simulink library "tandem_tiltwing_lib"  (R2018b)
settings: Solver=VariableStepAuto  StartTime=0.0  StopTime=10.0  RelTol=1e-3
undefined symbols (not defined in the file or in its folder): envir, euler2Quat, tiltwing
libraries: propulsion_lib x4, actuators_lib x3, simple_wing_lib x2, simpleFuselage_lib x1, ground_lib x1, rigidBody_lib x1
settings Model: Creator=Ybeyer  LastModifiedBy=yannic
settings SFSimCC: SimUseLocalCustomCode=off
settings RTWCC: RTWUseLocalCustomCode=off
settings CodeAppCC: StateflowObjectComments=on

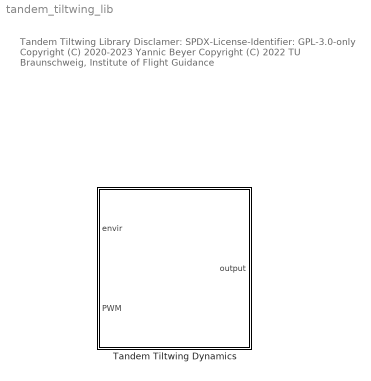
== system tandem_tiltwing_lib ==
  note: Tandem Tiltwing Library
      |
      | Disclamer:
      | SPDX-License-Identifier: GPL-3.0-only
      |
      | Copyright (C) 2020-2023 Yannic Beyer
      | Copyright (C) 2022 TU Braunschweig, Institute of Flight Guidance
  Tandem Tiltwing Dynamics : Subsystem  mask{tiltwing=tiltwing}
      mask prompts: tiltwing "tiltwing struct"
      mask DialogControl DescGroupVar Prompt: Tandem Tiltwing Dynamics
      mask DialogControl DescTextVar Prompt: For initializing the tiltwing struct see tandemTiltwingLoadParams.m

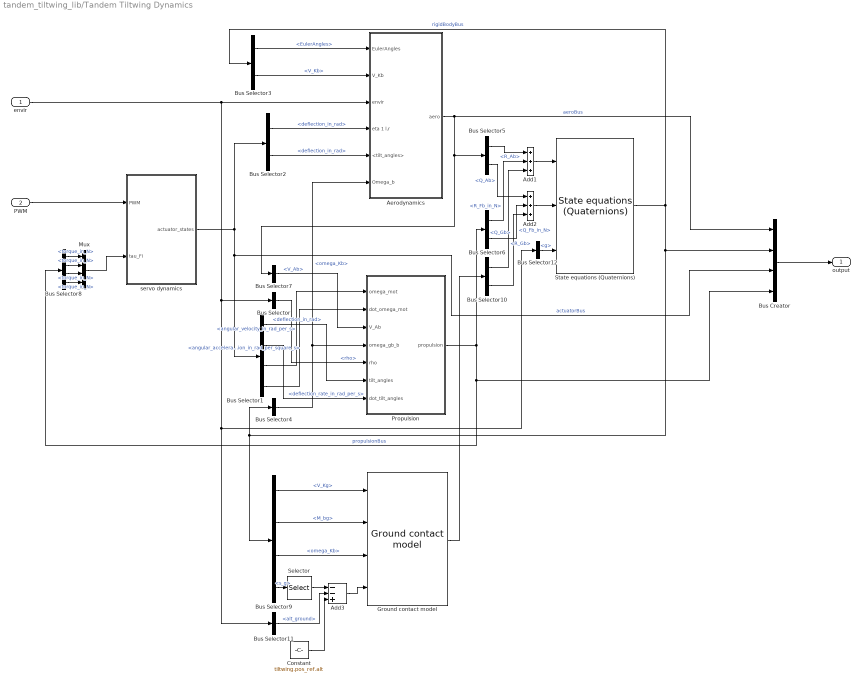
== system tandem_tiltwing_lib/Tandem Tiltwing Dynamics ==
  envir : Inport
  PWM : Inport  Port=2
  Add1 : Sum  Inputs=3
  Add2 : Sum  Inputs=3
  Add3 : Sum  Inputs=--+
  Aerodynamics : Subsystem
  Bus Creator : BusCreator  Inputs=4
  Bus Selector : BusSelector  OutputSignals=atmosphereBus.rho
  Bus Selector1 : BusSelector  OutputSignals=tilt_servos.deflection_in_rad,elevons.deflection_rate_in_rad_per_s,motors.angular_velocity_in_rad_per_s,motors.angular_acceleration_in_rad_per_square_s
  Bus Selector10 : BusSelector  OutputSignals=forces_and_moments.R_Gb,forces_and_moments.Q_Gb
  Bus Selector11 : BusSelector  OutputSignals=alt_ground
  Bus Selector12 : BusSelector  OutputSignals=g
  Bus Selector2 : BusSelector  OutputSignals=elevons.deflection_in_rad,tilt_servos.deflection_in_rad
  Bus Selector3 : BusSelector  OutputSignals=EulerAngles,V_Kb
  Bus Selector4 : BusSelector  OutputSignals=omega_Kb
  Bus Selector5 : BusSelector  OutputSignals=cg aerodynamics.R_Ab,cg aerodynamics.Q_Ab
  Bus Selector6 : BusSelector  OutputSignals=R_Fb_in_N,Q_Fb_in_N
  Bus Selector7 : BusSelector  OutputSignals=cg aerodynamics.aeroAxes.V_Ab
  Bus Selector8 : BusSelector  OutputSignals=propeller_1.torque_in_N,propeller_2.torque_in_N,propeller_3.torque_in_N,propeller_4.torque_in_N
  Bus Selector9 : BusSelector  OutputSignals=V_Kg,M_bg,omega_Kb,s_g
  Constant : Constant  Value=tiltwing.pos_ref.alt  VectorParams1D=off
  Ground contact model : ground_lib/Ground contact model  m=tiltwing.body.m  a_max=30  xyz_c_hit=tiltwing.config.collision_points_c  xyz_c_cg=tiltwing.config.xyz_c_cg  ground_softness_param=1e-5  k_h=1000  k_dot_h=100  mu=1  k_V=10
      settings: SourceProductName=LADAC
  Mux : Mux
  Propulsion : Subsystem
  Selector : Selector  InputPortWidth=3  IndexOptions=Index vector (dialog)  Indices=3  OutputSizes=1
  State equations (Quaternions) : rigidBody_lib/State equations (Quaternions)  m=tiltwing.body.m  I=tiltwing.body.I  is_g_checked=on  g=envir.g  omega_Kb_0=[ tiltwing.ic.p; tiltwing.ic.q; tiltwing.ic.r ]  q_bg_0=euler2Quat( [ tiltwing.ic.Phi; tiltwing.ic.Theta; tiltwing.ic.Psi ] )  V_Kb_0=[ tiltwing.ic.u; tiltwing.ic.v ; tiltwing.ic.w ]  s_g_0=[ tiltwing.ic.x; tiltwing.ic.y; tiltwing.ic.z ]
      settings: SourceProductName=LADAC
  servo dynamics : Subsystem
  output : Outport
  wires:
  PWM/1 -> servo dynamics/1(PWM)
  Bus Selector/1 -> Propulsion/5(rho)  "<rho>"
  servo dynamics/1(actuator_states) -> Bus Creator/3, Bus Selector1/1, Bus Selector2/1  "actuatorBus"
  Bus Selector1/1 -> Propulsion/6(tilt_angles)  "<deflection_in_rad>"
  Bus Selector1/3 -> Propulsion/1(omega_mot)  "<angular_velocity_in_rad_per_s>"
  Bus Selector1/4 -> Propulsion/2(dot_omega_mot)  "<angular_acceleration_in_rad_per_square_s>"
  Bus Selector2/1 -> Aerodynamics/4(eta 1 l,r)  "<deflection_in_rad>"
  Bus Selector2/2 -> Aerodynamics/5(<tilt_angles>)  "<deflection_in_rad>"
  State equations (Quaternions)/1 -> Bus Selector3/1, Bus Selector9/1, Bus Selector4/1, Bus Creator/2  "rigidBodyBus"
  Bus Selector3/2 -> Aerodynamics/2(V_Kb)  "<V_Kb>"
  Bus Selector3/1 -> Aerodynamics/1("EulerAngles ")  "<EulerAngles>"
  Bus Selector4/1 -> Propulsion/4("omega_gb_b "), Aerodynamics/6(Omega_b)  "<omega_Kb>"
  Bus Selector5/1 -> Add1/1  "<R_Ab>"
  Bus Selector5/2 -> Add2/1  "<Q_Ab>"
  Aerodynamics/1(aero) -> Bus Creator/1, Bus Selector5/1, Bus Selector7/1  "aeroBus"
  Bus Selector6/2 -> Add2/2  "<Q_Fb_in_N>"
  Bus Selector6/1 -> Add1/2  "<R_Fb_in_N>"
  Propulsion/1(propulsion) -> Bus Creator/4, Bus Selector8/1, Bus Selector6/1  "propulsionBus"
  Bus Selector7/1 -> Propulsion/3(V_Ab)  "<V_Ab>"
  Bus Selector9/1 -> Ground contact model/1  "<V_Kg>"
  Add1/1 -> State equations (Quaternions)/1
  Add2/1 -> State equations (Quaternions)/2
  Bus Selector9/3 -> Ground contact model/3  "<omega_Kb>"
  Bus Selector9/2 -> Ground contact model/2  "<M_bg>"
  Ground contact model/1 -> Bus Selector10/1
  Bus Selector10/1 -> Add1/3  "<R_Gb>"
  Bus Selector9/4 -> Selector/1  "<s_g>"
  Add3/1 -> Ground contact model/4
  Bus Selector11/1 -> Add3/2  "<alt_ground>"
  Selector/1 -> Add3/1
  Bus Selector10/2 -> Add2/3  "<Q_Gb>"
  Bus Selector1/2 -> Propulsion/7(dot_tilt_angles)  "<deflection_rate_in_rad_per_s>"
  Bus Selector8/4 -> Mux/4  "<torque_in_N>"
  Bus Selector8/3 -> Mux/3  "<torque_in_N>"
  Bus Selector8/2 -> Mux/2  "<torque_in_N>"
  Bus Selector8/1 -> Mux/1  "<torque_in_N>"
  Mux/1 -> servo dynamics/2(tau_Fi)
  Bus Creator/1 -> output/1
  envir/1 -> Aerodynamics/3(envir), Bus Selector/1, Bus Selector11/1, Bus Selector12/1
  Constant/1 -> Add3/3
  Bus Selector12/1 -> State equations (Quaternions)/3  "<g>"

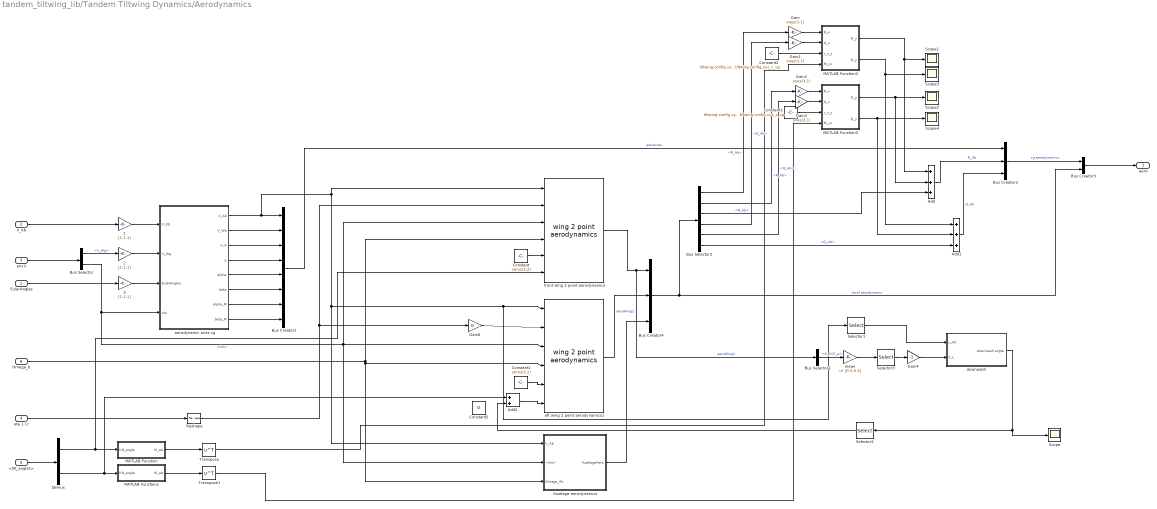
== system tandem_tiltwing_lib/Tandem Tiltwing Dynamics/Aerodynamics ==
  "EulerAngles " : Inport
  V_Kb : Inport  Port=2
  envir : Inport  Port=3
  eta 1 l,r : Inport  Port=4
  <tilt_angles> : Inport  Port=5
  Omega_b : Inport  Port=6
  1 : Gain  Gain=[1;1;1]
  2 : Gain  Gain=[1;1;1]  OutDataTypeStr=double
  3 : Gain  Gain=[1;1;1]
  Add : Sum  Inputs=+++
  Add1 : Sum  Inputs=+++
  Add2 : Sum
  Bus Creator1 : BusCreator  Inputs=8
  Bus Creator2 : BusCreator  Inputs=3
  Bus Creator3 : BusCreator  Inputs=2
  Bus Creator4 : BusCreator  Inputs=3
  Bus Selector : BusSelector  OutputSignals=windBus.V_Wg,atmosphereBus.rho
  Bus Selector1 : BusSelector  OutputSignals=dynamics.C_XYZ_a
  Bus Selector2 : BusSelector  OutputSignals=aeroWing1.dynamics.R_Ab,aeroWing2.dynamics.R_Ab,aeroFuselage.dynamics.R_Ab,aeroWing1.dynamics.Q_Ab,aeroWing2.dynamics.Q_Ab,aeroFuselage.dynamics.Q_Ab
  Constant : Constant  Value=zeros(3,2)
  Constant1 : Constant  Value=zeros(3,2)
  Constant2 : Constant  Value=tiltwing.config.xyz_c_tp1-tiltwing.config.xyz_c_cg
  Constant3 : Constant  Value=tiltwing.config.xyz_c_tp2-tiltwing.config.xyz_c_cg
  Constant5 : Constant  Value=0
  Demux : Demux  Outputs=2
  Gain{,1..3} (4 alike) : Gain  Gain=ones(3,1)
  Gain4 : Gain  Gain=-1
  Gain6 : Gain  Gain=0
  MATLAB Function : MATLAB Function  TreatAsAtomicUnit=on
  MATLAB Function1 : MATLAB Function  TreatAsAtomicUnit=on
  MATLAB Function2 : MATLAB Function  TreatAsAtomicUnit=on
  MATLAB Function3 : MATLAB Function  TreatAsAtomicUnit=on
  Reshape : Reshape  OutputDimensionality=Row vector (2-D)
  Scope{,1..4} (5 alike) : Scope
  Selector1 : Selector  InputPortWidth=3  IndexOptions=Index vector (dialog)  Indices=1  OutputSizes=1
  Selector2 : Selector  InputPortWidth=1  IndexOptions=Index vector (dialog)  Indices=1  OutputSizes=1
  Selector3 : Selector  InputPortWidth=3  IndexOptions=Index vector (dialog)  Indices=3  OutputSizes=1
  Transpose : Math  Operator=transpose  SaturateOnIntegerOverflow=on
  Transpose1 : Math  Operator=transpose  SaturateOnIntegerOverflow=on
  aerodynamic axes cg : MATLAB Function  TreatAsAtomicUnit=on
  aft wing 2 point aerodynamics1 : simple_wing_lib/wing 2 point aerodynamics  wingStruct=tiltwing.aero.wing_2  xyz_wing_c=tiltwing.config.xyz_c_tp2  xyz_cg_c=tiltwing.config.xyz_c_cg
      settings: SourceProductName=LADAC
  downwash : Subsystem
  front wing 2 point aerodynamics : simple_wing_lib/wing 2 point aerodynamics  wingStruct=tiltwing.aero.wing_1  xyz_wing_c=tiltwing.config.xyz_c_tp1  xyz_cg_c=tiltwing.config.xyz_c_cg
      settings: SourceProductName=LADAC
  fuselage aerodynamics : Subsystem
  mean : Gain  Gain=[0.5;0.5]  Multiplication=Matrix(u*K)
  aero : Outport
  wires:
  envir/1 -> Bus Selector/1
  Bus Selector/1 -> 2/1  "<V_Wg>"
  2/1 -> aerodynamic axes cg/2(V_Wg)
  "EulerAngles "/1 -> 3/1
  1/1 -> aerodynamic axes cg/1(V_Kb)
  V_Kb/1 -> 1/1
  3/1 -> aerodynamic axes cg/3(EulerAngles)
  Bus Selector/2 -> aft wing 2 point aerodynamics1/3, fuselage aerodynamics/2(<rho>), front wing 2 point aerodynamics/3, aerodynamic axes cg/4(rho)  "<rho>"
  eta 1 l,r/1 -> Reshape/1
  aerodynamic axes cg/2(V_Wb) -> Bus Creator1/2
  aerodynamic axes cg/3(V_A) -> Bus Creator1/3
  aerodynamic axes cg/4(q) -> Bus Creator1/4
  aerodynamic axes cg/5(alpha) -> Bus Creator1/5
  aerodynamic axes cg/6(beta) -> Bus Creator1/6
  aerodynamic axes cg/7(alpha_M) -> Bus Creator1/7
  aerodynamic axes cg/8(beta_M) -> Bus Creator1/8
  Bus Creator1/1 -> Bus Creator2/1  "aeroAxes"
  Bus Creator2/1 -> Bus Creator3/1  "cg aerodynamics"
  Bus Creator4/1 -> Bus Creator3/2, Bus Selector2/1  "local aerodynamic"
  Bus Creator3/1 -> aero/1
  front wing 2 point aerodynamics/1 -> Bus Selector1/1, Bus Creator4/1  "aeroWing1"
  aft wing 2 point aerodynamics1/1 -> Bus Creator4/2  "aeroWing2"
  fuselage aerodynamics/1(fuselageAero) -> Bus Creator4/3
  Bus Selector2/3 -> Add/3  "<R_Ab>"
  Bus Selector2/2 -> Gain2/1  "<R_Ab>"
  Bus Selector2/1 -> Gain/1  "<R_Ab>"
  Bus Selector2/6 -> Add1/3  "<Q_Ab>"
  Bus Selector2/5 -> Gain3/1  "<Q_Ab>"
  Bus Selector2/4 -> Gain1/1  "<Q_Ab>"
  Add/1 -> Bus Creator2/2  "R_Ab"
  Add1/1 -> Bus Creator2/3  "Q_Ab"
  Constant/1 -> front wing 2 point aerodynamics/5
  Constant1/1 -> aft wing 2 point aerodynamics1/5
  <tilt_angles>/1 -> Demux/1
  Demux/1 -> MATLAB Function/1(tilt_angle), front wing 2 point aerodynamics/6
  Demux/2 -> MATLAB Function1/1(tilt_angle), Add2/1
  aerodynamic axes cg/1(V_Ab) -> Bus Creator1/1, front wing 2 point aerodynamics/1, fuselage aerodynamics/1(V_Ab), Selector1/1, aft wing 2 point aerodynamics1/1
  MATLAB Function1/1(M_wb) -> Transpose1/1
  MATLAB Function/1(M_wb) -> Transpose/1
  Omega_b/1 -> front wing 2 point aerodynamics/4, fuselage aerodynamics/3(Omega_Ab), aft wing 2 point aerodynamics1/4
  Constant2/1 -> MATLAB Function2/3(r_x_y)
  Constant3/1 -> MATLAB Function3/3(r_x_y)
  MATLAB Function2/1(R_y) -> Scope1/1, Add/1
  MATLAB Function3/1(R_y) -> Scope2/1, Add/2
  MATLAB Function2/2(Q_y) -> Scope3/1, Add1/1
  MATLAB Function3/2(Q_y) -> Add1/2, Scope4/1
  Gain/1 -> MATLAB Function2/1(R_x)
  Gain1/1 -> MATLAB Function2/2(Q_x)
  Gain2/1 -> MATLAB Function3/1(R_x)
  Gain3/1 -> MATLAB Function3/2(Q_x)
  Transpose/1 -> MATLAB Function2/4(M_yx)
  Transpose1/1 -> MATLAB Function3/4(M_yx)
  Add2/1 -> aft wing 2 point aerodynamics1/6
  downwash/1(downwash angle) -> Selector2/1, Scope/1
  Gain4/1 -> downwash/2(C_L)
  Selector1/1 -> downwash/1(u_Ab)
  Bus Selector1/1 -> mean/1  "<C_XYZ_a>"
  Selector2/1 -> Add2/2
  Selector3/1 -> Gain4/1
  mean/1 -> Selector3/1
  Reshape/1 -> Gain6/1, front wing 2 point aerodynamics/2
  Gain6/1 -> aft wing 2 point aerodynamics1/2

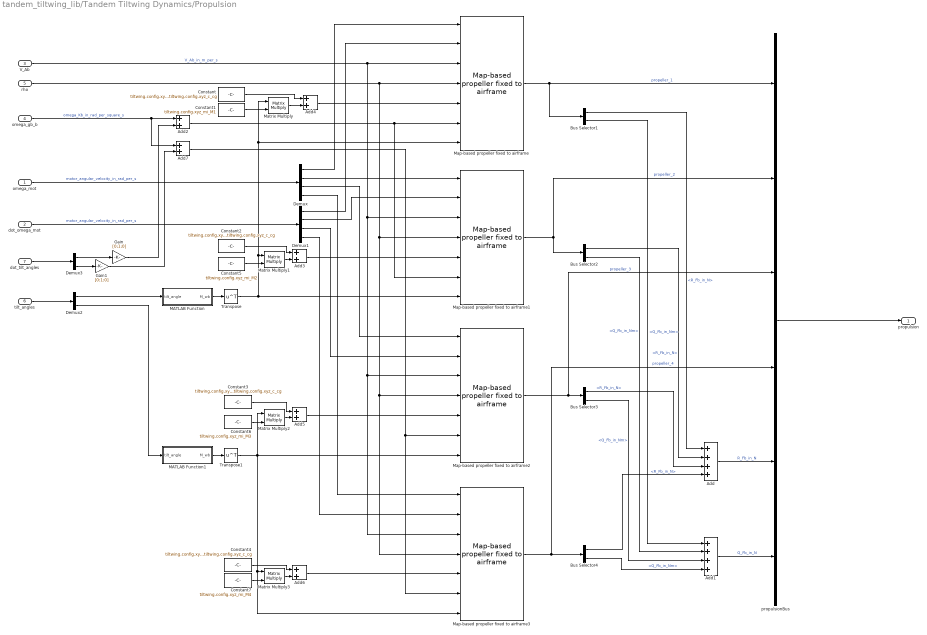
== system tandem_tiltwing_lib/Tandem Tiltwing Dynamics/Propulsion ==
  omega_mot : Inport  OutDataTypeStr=double  PortDimensions=4  SampleTime=0
  dot_omega_mot : Inport  Port=2  OutDataTypeStr=double  PortDimensions=4  SampleTime=0
  V_Ab : Inport  Port=3  OutDataTypeStr=double  PortDimensions=3  SampleTime=0
  "omega_gb_b " : Inport  Port=4  OutDataTypeStr=double  PortDimensions=3  SampleTime=0
  rho : Inport  Port=5  OutDataTypeStr=double  PortDimensions=1
  tilt_angles : Inport  Port=6
  dot_tilt_angles : Inport  Port=7
  Add : Sum  Inputs=4
  Add1 : Sum  Inputs=4
  Add{2..7} (6 alike) : Sum
  Bus Selector{1..4} (4 alike) : BusSelector  OutputSignals=R_Fb_in_N,Q_Fb_in_Nm
  Constant : Constant  Value=tiltwing.config.xyz_c_tp1-tiltwing.config.xyz_c_cg
  Constant1 : Constant  Value=tiltwing.config.xyz_mi_M1
  Constant2 : Constant  Value=tiltwing.config.xyz_c_tp1-tiltwing.config.xyz_c_cg
  Constant3 : Constant  Value=tiltwing.config.xyz_c_tp2-tiltwing.config.xyz_c_cg
  Constant4 : Constant  Value=tiltwing.config.xyz_c_tp2-tiltwing.config.xyz_c_cg
  Constant5 : Constant  Value=tiltwing.config.xyz_mi_M2
  Constant6 : Constant  Value=tiltwing.config.xyz_mi_M3
  Constant7 : Constant  Value=tiltwing.config.xyz_mi_M4
  Demux : Demux
  Demux1 : Demux
  Demux2 : Demux  Outputs=2
  Demux3 : Demux  Outputs=2
  Gain : Gain  Gain=[0;1;0]
  Gain1 : Gain  Gain=[0;1;0]
  MATLAB Function : MATLAB Function  TreatAsAtomicUnit=on
  MATLAB Function1 : MATLAB Function  TreatAsAtomicUnit=on
  Map-based propeller fixed to airframe : propulsion_lib/Map-based propeller fixed to airframe  prop_map_fit=prop.map_fit  I_prop=tiltwing.prop.I  rotation_orientation=tiltwing.config.propDir(1)
      settings: SourceProductName=LADAC
  Map-based propeller fixed to airframe1 : propulsion_lib/Map-based propeller fixed to airframe  prop_map_fit=prop.map_fit  I_prop=tiltwing.prop.I  rotation_orientation=tiltwing.config.propDir(2)
      settings: SourceProductName=LADAC
  Map-based propeller fixed to airframe2 : propulsion_lib/Map-based propeller fixed to airframe  prop_map_fit=prop.map_fit  I_prop=tiltwing.prop.I  rotation_orientation=tiltwing.config.propDir(3)
      settings: SourceProductName=LADAC
  Map-based propeller fixed to airframe3 : propulsion_lib/Map-based propeller fixed to airframe  prop_map_fit=prop.map_fit  I_prop=tiltwing.prop.I  rotation_orientation=tiltwing.config.propDir(4)
      settings: SourceProductName=LADAC
  Matrix Multiply{,1..3} (4 alike) : Product  Multiplication=Matrix(*)
  Transpose : Math  Operator=transpose  SaturateOnIntegerOverflow=on
  Transpose1 : Math  Operator=transpose  SaturateOnIntegerOverflow=on
  propulsionBus : BusCreator  Inputs=6
  propulsion : Outport  SampleTime=0
  wires:
  Demux1/1 -> Map-based propeller fixed to airframe/2
  V_Ab/1 -> Map-based propeller fixed to airframe3/3, Map-based propeller fixed to airframe2/3, Map-based propeller fixed to airframe1/3, Map-based propeller fixed to airframe/3  "V_Ab_in_m_per_s"
  Bus Selector1/1 -> Add/1  "<R_Fb_in_N>"
  Add4/1 -> Map-based propeller fixed to airframe/5
  Bus Selector2/1 -> Add/2  "<R_Fb_in_N>"
  Bus Selector1/2 -> Add1/1  "<Q_Fb_in_Nm>"
  Demux1/3 -> Map-based propeller fixed to airframe2/2
  Demux1/4 -> Map-based propeller fixed to airframe3/2
  Bus Selector4/1 -> Add/4  "<R_Fb_in_N>"
  Bus Selector3/2 -> Add1/3  "<Q_Fb_in_Nm>"
  Demux1/2 -> Map-based propeller fixed to airframe1/2
  Demux/1 -> Map-based propeller fixed to airframe/1
  Add3/1 -> Map-based propeller fixed to airframe1/5
  Map-based propeller fixed to airframe3/1 -> Bus Selector4/1, propulsionBus/4  "propeller_4"
  propulsionBus/1 -> propulsion/1
  Bus Selector4/2 -> Add1/4  "<Q_Fb_in_Nm>"
  Demux/2 -> Map-based propeller fixed to airframe1/1
  Map-based propeller fixed to airframe1/1 -> Bus Selector2/1, propulsionBus/2  "propeller_2"
  Bus Selector3/1 -> Add/3  "<R_Fb_in_N>"
  Transpose1/1 -> Map-based propeller fixed to airframe2/7, Matrix Multiply3/1, Map-based propeller fixed to airframe3/7, Matrix Multiply2/1
  Add/1 -> propulsionBus/5  "R_Fb_in_N"
  Add2/1 -> Map-based propeller fixed to airframe1/6, Map-based propeller fixed to airframe/6
  Add5/1 -> Map-based propeller fixed to airframe2/5
  rho/1 -> Map-based propeller fixed to airframe3/4, Map-based propeller fixed to airframe2/4, Map-based propeller fixed to airframe1/4, Map-based propeller fixed to airframe/4
  Map-based propeller fixed to airframe2/1 -> propulsionBus/3, Bus Selector3/1  "propeller_3"
  Demux/3 -> Map-based propeller fixed to airframe2/1
  Transpose/1 -> Matrix Multiply1/1, Matrix Multiply/1, Map-based propeller fixed to airframe/7, Map-based propeller fixed to airframe1/7
  Bus Selector2/2 -> Add1/2  "<Q_Fb_in_Nm>"
  Map-based propeller fixed to airframe/1 -> propulsionBus/1, Bus Selector1/1  "propeller_1"
  Add1/1 -> propulsionBus/6  "Q_Fb_in_N"
  Add6/1 -> Map-based propeller fixed to airframe3/5
  Demux/4 -> Map-based propeller fixed to airframe3/1
  omega_mot/1 -> Demux/1  "motor_angular_velocity_in_rad_per_s"
  dot_omega_mot/1 -> Demux1/1  "motor_angular_velocity_in_rad_per_s"
  MATLAB Function/1(M_wb) -> Transpose/1
  tilt_angles/1 -> Demux2/1
  Demux2/1 -> MATLAB Function/1(tilt_angle)
  MATLAB Function1/1(M_wb) -> Transpose1/1
  Demux2/2 -> MATLAB Function1/1(tilt_angle)
  dot_tilt_angles/1 -> Demux3/1
  Gain/1 -> Add2/2
  "omega_gb_b "/1 -> Add7/1, Add2/1  "omega_Kb_in_rad_per_square_s"
  Constant2/1 -> Add3/1
  Constant/1 -> Add4/1
  Constant3/1 -> Add5/1
  Constant4/1 -> Add6/1
  Demux3/1 -> Gain/1
  Demux3/2 -> Gain1/1
  Gain1/1 -> Add7/2
  Add7/1 -> Map-based propeller fixed to airframe3/6, Map-based propeller fixed to airframe2/6
  Matrix Multiply/1 -> Add4/2
  Constant1/1 -> Matrix Multiply/2
  Matrix Multiply1/1 -> Add3/2
  Constant5/1 -> Matrix Multiply1/2
  Matrix Multiply2/1 -> Add5/2
  Constant6/1 -> Matrix Multiply2/2
  Matrix Multiply3/1 -> Add6/2
  Constant7/1 -> Matrix Multiply3/2

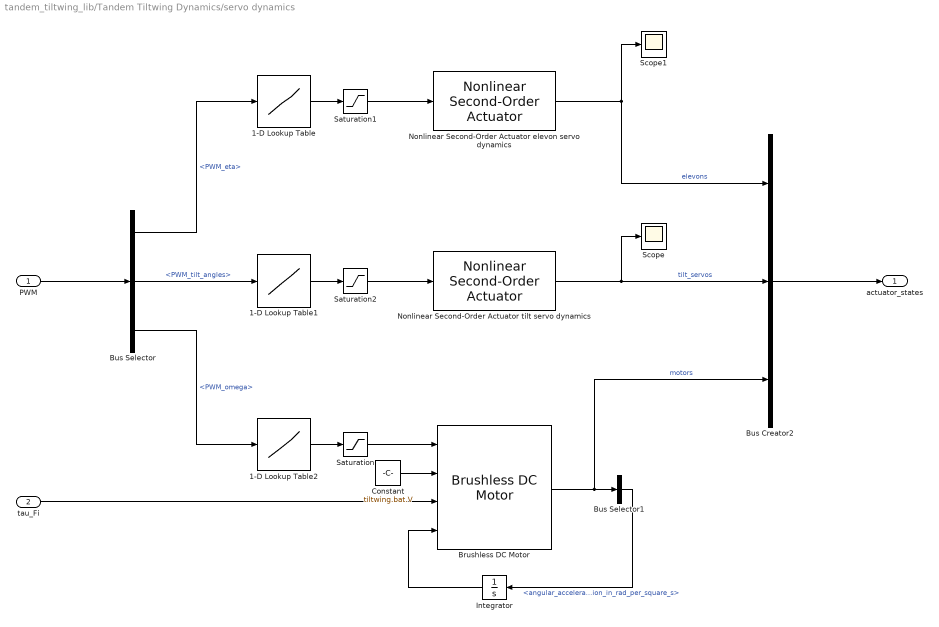
== system tandem_tiltwing_lib/Tandem Tiltwing Dynamics/servo dynamics ==
  PWM : Inport
  tau_Fi : Inport  Port=2
  1-D Lookup Table : Lookup_n-D  NumberOfTableDimensions=1  BreakpointsForDimension1=[1000;2000]  Table=[tiltwing.act.elevon.deflectionMin;tiltwing.act.elevon.deflectionMax]  InternalRulePriority=Speed  RndMeth=Simplest  InputSameDT=on
  1-D Lookup Table1 : Lookup_n-D  NumberOfTableDimensions=1  BreakpointsForDimension1=[900;2100]  Table=[tiltwing.act.tilt.deflectionMin;tiltwing.act.tilt.deflectionMax]  InternalRulePriority=Speed  RndMeth=Simplest  InputSameDT=on
  1-D Lookup Table2 : Lookup_n-D  NumberOfTableDimensions=1  BreakpointsForDimension1=[1000;2000]  Table=[0;1]  InternalRulePriority=Speed  RndMeth=Simplest  InputSameDT=on
  Brushless DC Motor : actuators_lib/Brushless DC Motor  K_T=tiltwing.motor.KT  J_prop=tiltwing.prop.I  R_i=tiltwing.motor.R  IC_omega=tiltwing.ic.omega  omega_max=Inf  omega_min=0
      settings: SourceProductName=LADAC
  Bus Creator2 : BusCreator  Inputs=3
  Bus Selector : BusSelector  OutputSignals=PWM_eta,PWM_tilt_angles,PWM_omega
  Bus Selector1 : BusSelector  OutputSignals=angular_acceleration_in_rad_per_square_s
  Constant : Constant  Value=tiltwing.bat.V
  Integrator : Integrator  InitialCondition=tiltwing.ic.omega  ContinuousStateAttributes='omega_i'
  Nonlinear Second-Order Actuator elevon servo dynamics : actuators_lib/Nonlinear Second-Order Actuator  omega=tiltwing.act.elevon.naturalFrequency  d=tiltwing.act.elevon.dampingRatio  A_max=tiltwing.act.elevon.deflectionMax  A_min=tiltwing.act.elevon.deflectionMin  dot_A_max=tiltwing.act.elevon.deflectionRateMax  dot_A_min=-tiltwing.act.elevon.deflectionRateMax  A_0=deg2rad([tiltwing.ic.elevon_1;tiltwing.ic.elevon_2])  dot_A_0=[0;0]
      settings: SourceProductName=LADAC
  Nonlinear Second-Order Actuator tilt servo dynamics : actuators_lib/Nonlinear Second-Order Actuator  omega=tiltwing.act.tilt.naturalFrequency  d=tiltwing.act.tilt.dampingRatio  A_max=tiltwing.act.tilt.deflectionMax  A_min=tiltwing.act.tilt.deflectionMin  dot_A_max=tiltwing.act.tilt.deflectionRateMax  dot_A_min=-tiltwing.act.tilt.deflectionRateMax  A_0=deg2rad([tiltwing.ic.tilt_angle_1;tiltwing.ic.tilt_angle_2])  dot_A_0=[0;0]
      settings: SourceProductName=LADAC
  Saturation : Saturate  UpperLimit=1  LowerLimit=0
  Saturation1 : Saturate  UpperLimit=tiltwing.act.elevon.deflectionMax  LowerLimit=tiltwing.act.elevon.deflectionMin
  Saturation2 : Saturate  UpperLimit=tiltwing.act.tilt.deflectionMax  LowerLimit=tiltwing.act.tilt.deflectionMin
  Scope : Scope
  Scope1 : Scope
  actuator_states : Outport
  wires:
  Bus Selector1/1 -> Integrator/1  "<angular_acceleration_in_rad_per_square_s>"
  tau_Fi/1 -> Brushless DC Motor/3
  Saturation/1 -> Brushless DC Motor/1
  Saturation2/1 -> Nonlinear Second-Order Actuator tilt servo dynamics/1
  1-D Lookup Table/1 -> Saturation1/1
  1-D Lookup Table1/1 -> Saturation2/1
  Saturation1/1 -> Nonlinear Second-Order Actuator elevon servo dynamics/1
  1-D Lookup Table2/1 -> Saturation/1
  PWM/1 -> Bus Selector/1
  Bus Selector/1 -> 1-D Lookup Table/1  "<PWM_eta>"
  Bus Selector/2 -> 1-D Lookup Table1/1  "<PWM_tilt_angles>"
  Bus Selector/3 -> 1-D Lookup Table2/1  "<PWM_omega>"
  Bus Creator2/1 -> actuator_states/1
  Nonlinear Second-Order Actuator tilt servo dynamics/1 -> Bus Creator2/2, Scope/1  "tilt_servos"
  Nonlinear Second-Order Actuator elevon servo dynamics/1 -> Bus Creator2/1, Scope1/1  "elevons"
  Brushless DC Motor/1 -> Bus Creator2/3, Bus Selector1/1  "motors"
  Constant/1 -> Brushless DC Motor/2
  Integrator/1 -> Brushless DC Motor/4

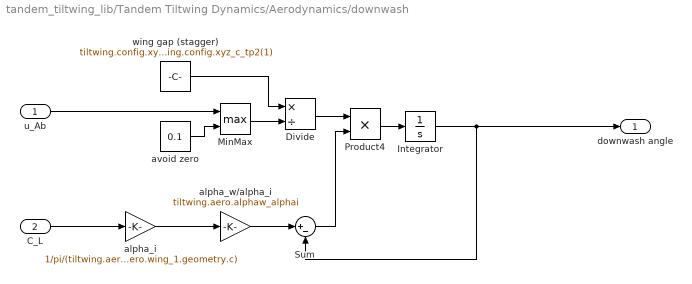
== system tandem_tiltwing_lib/Tandem Tiltwing Dynamics/Aerodynamics/downwash ==
  u_Ab : Inport
  C_L : Inport  Port=2
  Divide : Product  Inputs=*/
  Integrator : Integrator  ContinuousStateAttributes='downwash'
  MinMax : MinMax  Function=max  Inputs=2
  Product4 : Product
  Sum : Sum  Inputs=|+-
  alpha_i : Gain  Gain=1/pi/(tiltwing.aero.wing_1.geometry.b/tiltwing.aero.wing_1.geometry.c)
  alpha_w/alpha_i : Gain  Gain=tiltwing.aero.alphaw_alphai
  avoid zero : Constant  Value=0.1
  wing gap (stagger) : Constant  Value=tiltwing.config.xyz_c_tp1(1)-tiltwing.config.xyz_c_tp2(1)
  downwash angle : Outport  PortDimensions=1
  wires:
  alpha_i/1 -> alpha_w/alpha_i/1
  alpha_w/alpha_i/1 -> Sum/1
  Divide/1 -> Product4/1
  wing gap (stagger)/1 -> Divide/1
  MinMax/1 -> Divide/2
  avoid zero/1 -> MinMax/2
  u_Ab/1 -> MinMax/1
  C_L/1 -> alpha_i/1
  Integrator/1 -> Sum/2, downwash angle/1
  Product4/1 -> Integrator/1
  Sum/1 -> Product4/2

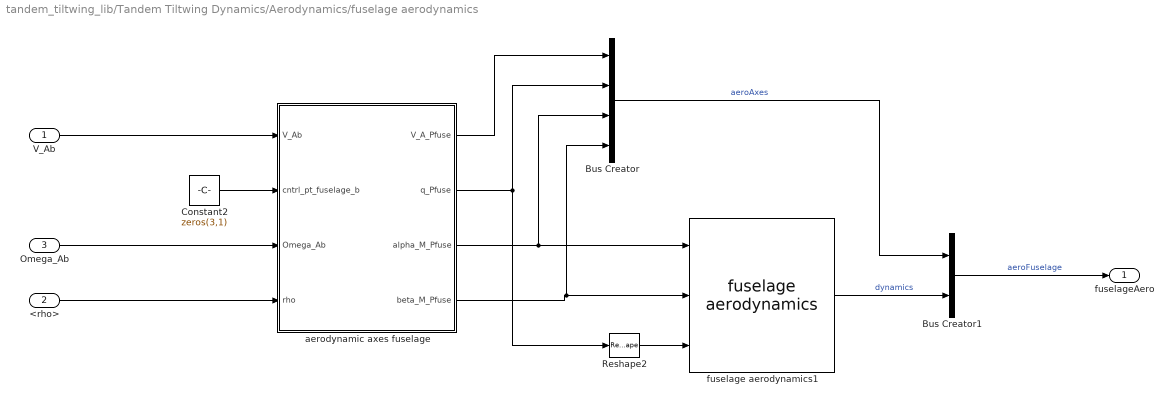
== system tandem_tiltwing_lib/Tandem Tiltwing Dynamics/Aerodynamics/fuselage aerodynamics ==
  V_Ab : Inport
  <rho> : Inport  Port=2
  Omega_Ab : Inport  Port=3
  Bus Creator : BusCreator  Inputs=4
  Bus Creator1 : BusCreator  Inputs=2
  Constant2 : Constant  Value=zeros(3,1)
  Reshape2 : Reshape  OutputDimensionality=Row vector (2-D)
  aerodynamic axes fuselage : MATLAB Function  TreatAsAtomicUnit=on
  fuselage aerodynamics1 : simpleFuselage_lib/fuselage aerodynamics  simple_fuselage=tiltwing.aero.fuselage
      settings: SourceProductName=LADAC
  fuselageAero : Outport
  wires:
  aerodynamic axes fuselage/3(alpha_M_Pfuse) -> fuselage aerodynamics1/1, Bus Creator/3
  Constant2/1 -> aerodynamic axes fuselage/2(cntrl_pt_fuselage_b)
  Reshape2/1 -> fuselage aerodynamics1/3
  aerodynamic axes fuselage/4(beta_M_Pfuse) -> fuselage aerodynamics1/2, Bus Creator/4
  Omega_Ab/1 -> aerodynamic axes fuselage/3(Omega_Ab)
  V_Ab/1 -> aerodynamic axes fuselage/1(V_Ab)
  aerodynamic axes fuselage/1(V_A_Pfuse) -> Bus Creator/1
  <rho>/1 -> aerodynamic axes fuselage/4(rho)
  aerodynamic axes fuselage/2(q_Pfuse) -> Reshape2/1, Bus Creator/2
  Bus Creator/1 -> Bus Creator1/1  "aeroAxes"
  fuselage aerodynamics1/1 -> Bus Creator1/2  "dynamics"
  Bus Creator1/1 -> fuselageAero/1  "aeroFuselage"

== matlab function tandem_tiltwing_lib/Tandem Tiltwing Dynamics/Aerodynamics/MATLAB Function ==
  data: tilt_angle input; M_wb output
function M_wb = fcn(tilt_angle)

cos_t = cos(tilt_angle);
sin_t = sin(tilt_angle);

M_wb = [ ...
    cos_t,  0,  -sin_t; ...
    0,      1,  0; ...
    sin_t,  0,  cos_t ...
    ];

end

== matlab function tandem_tiltwing_lib/Tandem Tiltwing Dynamics/Aerodynamics/aerodynamic axes cg ==
  data: V_Kb input; V_Ab output; V_Wb output; V_A output; q output; alpha output; beta output; V_Wg input; EulerAngles input; alpha_M output; beta_M output; rho input
function [ V_Ab, V_Wb, V_A, q, alpha, beta, alpha_M, beta_M ] = ...
    fcn( V_Kb, V_Wg, EulerAngles, rho ) %#codegen

% compute rotation matrix from g to b frame
M_bg = euler2Dcm( EulerAngles );

% compute velocities
V_Wb = M_bg * V_Wg;
V_Ab = V_Kb - V_Wb;

% calculate aerodynamic speed (TAS) and dynamic pressure
V_A = norm( V_Ab, 2 );
q   = rho/2 * V_A^2;

% compute aerodynamic angles
[ alpha, beta ] = aeroAngles( V_Ab );

% compute modified aerodynamic angles
[ alpha_M, beta_M ] = aeroAnglesMod( V_Ab );
 
end

== matlab function tandem_tiltwing_lib/Tandem Tiltwing Dynamics/Propulsion/MATLAB Function ==
  data: tilt_angle input; M_wb output
function M_wb = fcn(tilt_angle)

cos_t = cos(tilt_angle);
sin_t = sin(tilt_angle);

M_wb = [ ...
    cos_t,  0,  -sin_t; ...
    0,      1,  0; ...
    sin_t,  0,  cos_t ...
    ];

end

== matlab function tandem_tiltwing_lib/Tandem Tiltwing Dynamics/Aerodynamics/fuselage aerodynamics/aerodynamic axes fuselage ==
  data: V_Ab input; cntrl_pt_fuselage_b input; Omega_Ab input; V_A_Pfuse output; q_Pfuse output; alpha_M_Pfuse output; beta_M_Pfuse output; rho input
function [ V_A_Pfuse, q_Pfuse, alpha_M_Pfuse, beta_M_Pfuse ] = fcn( V_Ab, ...
    cntrl_pt_fuselage_b, Omega_Ab, rho )
%#codegen

% compute inflow at specified points
V_Ab_Pfuse = velocityFromRot( V_Ab, Omega_Ab, cntrl_pt_fuselage_b );
V_A_Pfuse = real( sqrt(V_Ab_Pfuse(1,:).^2 + V_Ab_Pfuse(2,:).^2 + V_Ab_Pfuse(3,:).^2) );
q_Pfuse = rho/2 * V_A_Pfuse.^2;
[ alpha_M_Pfuse, beta_M_Pfuse ] = aeroAnglesMod( V_Ab_Pfuse );

end

== matlab function tandem_tiltwing_lib/Tandem Tiltwing Dynamics/Aerodynamics/MATLAB Function1 ==
  data: tilt_angle input; M_wb output
function M_wb = fcn(tilt_angle)

cos_t = cos(tilt_angle);
sin_t = sin(tilt_angle);

M_wb = [ ...
    cos_t,  0,  -sin_t; ...
    0,      1,  0; ...
    sin_t,  0,  cos_t ...
    ];

end

== matlab function tandem_tiltwing_lib/Tandem Tiltwing Dynamics/Propulsion/MATLAB Function1 ==
  data: tilt_angle input; M_wb output
function M_wb = fcn(tilt_angle)

cos_t = cos(tilt_angle);
sin_t = sin(tilt_angle);

M_wb = [ ...
    cos_t,  0,  -sin_t; ...
    0,      1,  0; ...
    sin_t,  0,  cos_t ...
    ];

end

== matlab function tandem_tiltwing_lib/Tandem Tiltwing Dynamics/Aerodynamics/MATLAB Function2 ==
  data: R_x input; R_y output; Q_x input; r_x_y input; M_yx input; Q_y output
function [ R_y, Q_y ] = fcn( R_x, Q_x, r_x_y, M_yx )

[ R_y, Q_y ] = forceMomentTransform( R_x, Q_x, r_x_y, M_yx );

end

== matlab function tandem_tiltwing_lib/Tandem Tiltwing Dynamics/Aerodynamics/MATLAB Function3 ==
  data: R_x input; R_y output; Q_x input; r_x_y input; M_yx input; Q_y output
function [ R_y, Q_y ] = fcn( R_x, Q_x, r_x_y, M_yx )

[ R_y, Q_y ] = forceMomentTransform( R_x, Q_x, r_x_y, M_yx );

end
